simulink model "IMU_Filter_Benchmarking"  (R2026a)
settings: Solver=VariableStepAuto  StopTime=10
libraries: dspstat3 x4, simulink x3
settings Model: Creator=root  LastModifiedBy=root

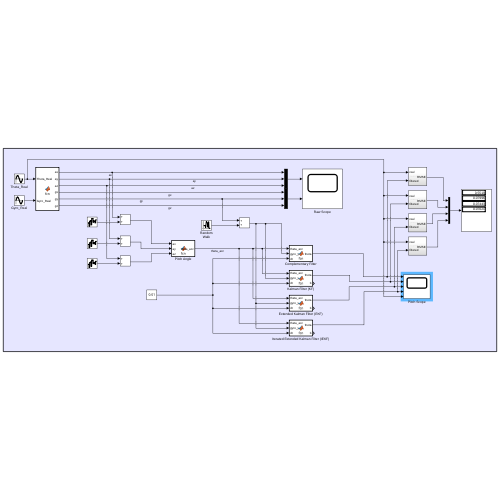
[thumbnail: Simulink's stored preview of the top-level diagram]
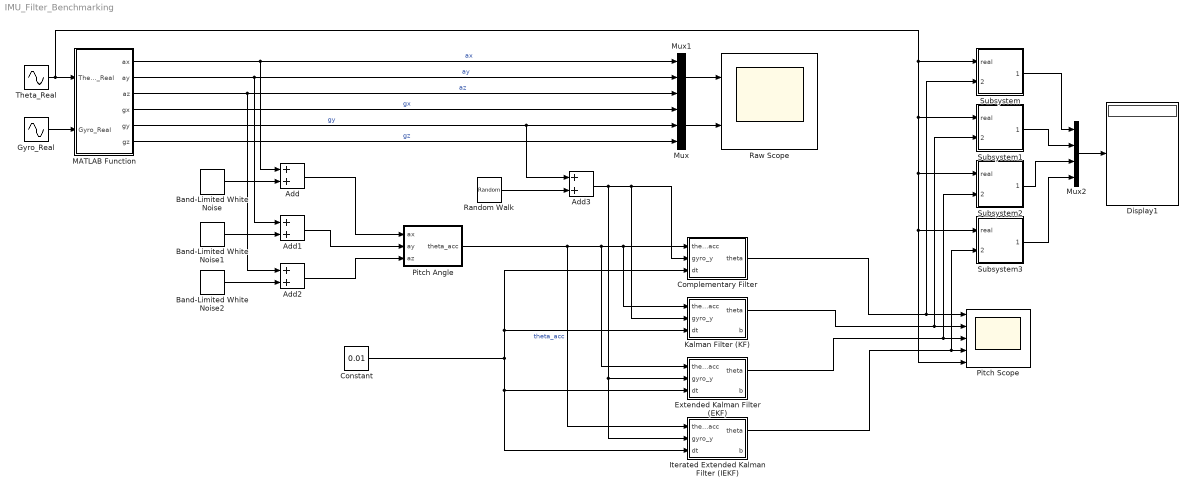
== system IMU_Filter_Benchmarking ==
  Add{,1..3} (4 alike) : Sum
  Band-Limited White Noise : simulink/Sources/Band-Limited White Noise  Cov=[0.1]  Ts=0.01  seed=[23341]
  Band-Limited White Noise1 : simulink/Sources/Band-Limited White Noise  Cov=[0.1]  Ts=0.01  seed=[24341]
  Band-Limited White Noise2 : simulink/Sources/Band-Limited White Noise  Cov=[0.1]  Ts=0.01  seed=[24741]
  Complementary Filter : MATLAB Function  TreatAsAtomicUnit=on
  Constant : Constant  Value=0.01
  Display1 : Display
  Extended Kalman Filter (EKF) : MATLAB Function  TreatAsAtomicUnit=on
  Gyro_Real : Sin  Amplitude=0.5  Phase=1.57  SampleTime=0
  Iterated Extended Kalman Filter (IEKF) : MATLAB Function  TreatAsAtomicUnit=on
  Kalman Filter (KF) : MATLAB Function  TreatAsAtomicUnit=on
  MATLAB Function : MATLAB Function  TreatAsAtomicUnit=on
  Mux : Mux  Inputs=3
  Mux1 : Mux  Inputs=3
  Mux2 : Mux
  Pitch Angle : MATLAB Function  TreatAsAtomicUnit=on
  Pitch Scope : Scope  NumInputPorts=5
      settings: ActiveDisplayYMinimum=-1.6362486288335127  ActiveDisplayYMaximum=1.8195667840554803
  Random Walk : RandomNumber  Mean=0.005  Variance=0.001  Seed=1324  SampleTime=0.01
  Raw Scope : Scope  NumInputPorts=2
      settings: ActiveDisplayYMinimum=-9.4165056943893433  ActiveDisplayYMaximum=14.411522746086121
  Subsystem : Subsystem
  Subsystem1 : Subsystem
  Subsystem2 : Subsystem
  Subsystem3 : Subsystem
  Theta_Real : Sin  Frequency=2.5  SampleTime=0
  wires:
  Iterated Extended Kalman Filter (IEKF)/1(theta) -> Subsystem3/2(filtered), Pitch Scope/4
  Extended Kalman Filter (EKF)/1(theta) -> Subsystem2/2(filtered), Pitch Scope/3
  Constant/1 -> Iterated Extended Kalman Filter (IEKF)/3(dt), Extended Kalman Filter (EKF)/3(dt), Kalman Filter (KF)/3(dt), Complementary Filter/3(dt)
  Complementary Filter/1(theta) -> Subsystem/2(filtered), Pitch Scope/1
  Mux1/1 -> Raw Scope/1
  Mux/1 -> Raw Scope/2
  MATLAB Function/1(ax) -> Mux1/1, Add/1  "ax"
  MATLAB Function/2(ay) -> Add1/1, Mux1/2  "ay"
  Pitch Angle/1(theta_acc) -> Extended Kalman Filter (EKF)/1(theta_acc), Kalman Filter (KF)/1(theta_acc), Complementary Filter/1(theta_acc), Iterated Extended Kalman Filter (IEKF)/1(theta_acc)  "theta_acc"
  Band-Limited White Noise1/1 -> Add1/2
  Band-Limited White Noise2/1 -> Add2/2
  Add3/1 -> Iterated Extended Kalman Filter (IEKF)/2(gyro_y), Extended Kalman Filter (EKF)/2(gyro_y), Kalman Filter (KF)/2(gyro_y), Complementary Filter/2(gyro_y)
  Add1/1 -> Pitch Angle/2(ay)
  Random Walk/1 -> Add3/2
  MATLAB Function/3(az) -> Add2/1, Mux1/3  "az"
  MATLAB Function/4(gx) -> Mux/1  "gx"
  MATLAB Function/6(gz) -> Mux/3  "gz"
  Kalman Filter (KF)/1(theta) -> Subsystem1/2(filtered), Pitch Scope/2
  Add/1 -> Pitch Angle/1(ax)
  MATLAB Function/5(gy) -> Add3/1, Mux/2  "gy"
  Band-Limited White Noise/1 -> Add/2
  Add2/1 -> Pitch Angle/3(az)
  Gyro_Real/1 -> MATLAB Function/2(Gyro_Real)
  Theta_Real/1 -> Subsystem/1(real), Subsystem1/1(real), Subsystem2/1(real), Subsystem3/1(real), Pitch Scope/5, MATLAB Function/1(Theta_Real)
  Subsystem/1(RMSE) -> Mux2/1
  Mux2/1 -> Display1/1
  Subsystem1/1(RMSE) -> Mux2/2
  Subsystem3/1(RMSE) -> Mux2/4
  Subsystem2/1(RMSE) -> Mux2/3

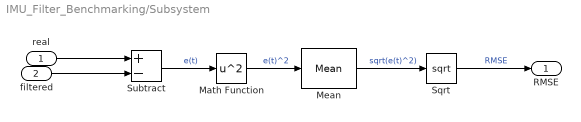
== system IMU_Filter_Benchmarking/Subsystem ==
  real : Inport
  filtered : Inport  Port=2
  Math Function : Math  Operator=square
  Mean : dspstat3/Mean  run=off  InputProcessing=Columns as channels (frame based)  reset_popup=None  directionMode=Each column  dimension=1  roiEnable=off  roiType=Rectangles  roiPortion=Entire ROI  roiOutput=Individual statistics for each ROI  roiFlag=off  roundingMode=Floor  overflowMode=off  outputDataTypeStr=Inherit: Same as accumulator  outputMin=[]  outputMax=[]  outputLastDataTypeStr=Inherit: Same as accumulator
  Sqrt : Sqrt
  Subtract : Sum  Inputs=+-
  RMSE : Outport
  wires:
  Math Function/1 -> Mean/1  "e(t)^2"
  Sqrt/1 -> RMSE/1  "RMSE"
  Mean/1 -> Sqrt/1  "sqrt(e(t)^2)"
  Subtract/1 -> Math Function/1  "e(t)"
  filtered/1 -> Subtract/2
  real/1 -> Subtract/1

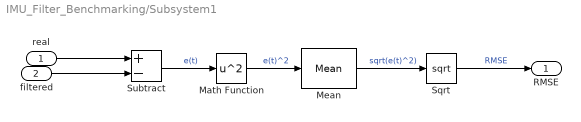
== system IMU_Filter_Benchmarking/Subsystem1 ==
  real : Inport
  filtered : Inport  Port=2
  Math Function : Math  Operator=square
  Mean : dspstat3/Mean  run=off  InputProcessing=Columns as channels (frame based)  reset_popup=None  directionMode=Each column  dimension=1  roiEnable=off  roiType=Rectangles  roiPortion=Entire ROI  roiOutput=Individual statistics for each ROI  roiFlag=off  roundingMode=Floor  overflowMode=off  outputDataTypeStr=Inherit: Same as accumulator  outputMin=[]  outputMax=[]  outputLastDataTypeStr=Inherit: Same as accumulator
  Sqrt : Sqrt
  Subtract : Sum  Inputs=+-
  RMSE : Outport
  wires:
  real/1 -> Subtract/1
  filtered/1 -> Subtract/2
  Subtract/1 -> Math Function/1  "e(t)"
  Mean/1 -> Sqrt/1  "sqrt(e(t)^2)"
  Sqrt/1 -> RMSE/1  "RMSE"
  Math Function/1 -> Mean/1  "e(t)^2"

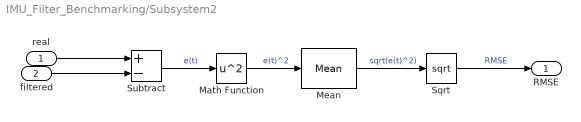
== system IMU_Filter_Benchmarking/Subsystem2 ==
  real : Inport
  filtered : Inport  Port=2
  Math Function : Math  Operator=square
  Mean : dspstat3/Mean  run=off  InputProcessing=Columns as channels (frame based)  reset_popup=None  directionMode=Each column  dimension=1  roiEnable=off  roiType=Rectangles  roiPortion=Entire ROI  roiOutput=Individual statistics for each ROI  roiFlag=off  roundingMode=Floor  overflowMode=off  outputDataTypeStr=Inherit: Same as accumulator  outputMin=[]  outputMax=[]  outputLastDataTypeStr=Inherit: Same as accumulator
  Sqrt : Sqrt
  Subtract : Sum  Inputs=+-
  RMSE : Outport
  wires:
  Math Function/1 -> Mean/1  "e(t)^2"
  Sqrt/1 -> RMSE/1  "RMSE"
  Mean/1 -> Sqrt/1  "sqrt(e(t)^2)"
  Subtract/1 -> Math Function/1  "e(t)"
  filtered/1 -> Subtract/2
  real/1 -> Subtract/1

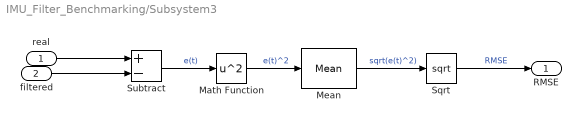
== system IMU_Filter_Benchmarking/Subsystem3 ==
  real : Inport
  filtered : Inport  Port=2
  Math Function : Math  Operator=square
  Mean : dspstat3/Mean  run=off  InputProcessing=Columns as channels (frame based)  reset_popup=None  directionMode=Each column  dimension=1  roiEnable=off  roiType=Rectangles  roiPortion=Entire ROI  roiOutput=Individual statistics for each ROI  roiFlag=off  roundingMode=Floor  overflowMode=off  outputDataTypeStr=Inherit: Same as accumulator  outputMin=[]  outputMax=[]  outputLastDataTypeStr=Inherit: Same as accumulator
  Sqrt : Sqrt
  Subtract : Sum  Inputs=+-
  RMSE : Outport
  wires:
  real/1 -> Subtract/1
  filtered/1 -> Subtract/2
  Subtract/1 -> Math Function/1  "e(t)"
  Mean/1 -> Sqrt/1  "sqrt(e(t)^2)"
  Sqrt/1 -> RMSE/1  "RMSE"
  Math Function/1 -> Mean/1  "e(t)^2"

== matlab function IMU_Filter_Benchmarking/Complementary Filter ==
  data: theta_acc input; theta output; gyro_y input; dt input
function theta = fcn(theta_acc, gyro_y, dt)
    theta_acc = double(theta_acc);
    gyro_y    = double(gyro_y);
    dt        = double(dt);

    % Set up the previous theta value
    persistent theta_prev
    if isempty(theta_prev)
        theta_prev = 0;
    end
    
    % Complementary filter w/ high-pass gyro + low-pass accelerometer
    alpha = 0.98;
    theta = alpha * (theta_prev + gyro_y * dt) + (1 - alpha) * theta_acc;
    theta_prev = theta;
end

== matlab function IMU_Filter_Benchmarking/Pitch Angle ==
  data: ax input; theta_acc output; ay input; az input
function theta_acc = fcn(ax, ay, az)
    % Calculate pitch angle in radians from static acceleration
    theta_acc = atan2(ax, sqrt(ay^2 + az^2));
end

== matlab function IMU_Filter_Benchmarking/Kalman Filter (KF) ==
  data: theta_acc input; theta output; gyro_y input; dt input; b output
function [theta, b] = fcn(theta_acc, gyro_y, dt)
    theta_acc = double(theta_acc);
    gyro_y    = double(gyro_y);
    dt        = double(dt);

    persistent x P
    if isempty(x)
        x = [0; 0];
        P = eye(2);
    end

    % --- EMPIRICAL COVARIANCE MATRICES ---
    R = 0.00000382;
    Q = [4.0e-10 , 0 ;
         0       , 1.0e-6];
    % ------------------------------------

    A = [1, -dt; 0, 1];
    B = [dt; 0];
    C = [1, 0];
    
    % Predict
    x_pred = A * x + B * gyro_y;
    P_pred = A * P * A' + Q;
    
    % Update
    K = (P_pred * C') / (C * P_pred * C' + R);
    x = x_pred + K * (theta_acc - C * x_pred);
    P = (eye(2) - K * C) * P_pred;
    
    % Clamp the angle back to [-pi, pi] interval after the state update
    x(1) = atan2(sin(x(1)), cos(x(1)));

    theta = x(1);
    b     = x(2);
end

== matlab function IMU_Filter_Benchmarking/Iterated Extended Kalman Filter (IEKF) ==
  data: theta_acc input; theta output; gyro_y input; dt input; b output
function [theta, b] = fcn(theta_acc, gyro_y, dt)
    theta_acc = double(theta_acc);
    gyro_y    = double(gyro_y);
    dt        = double(dt);

    persistent x P
    if isempty(x)
        x = [0; 0];
        P = eye(2);
    end

    % --- EMPIRICAL COVARIANCE MATRICES ---
    R = 0.00000382;
    Q = [4.0e-10 , 0 ;
         0       , 1.0e-6];
    % ------------------------------------

    A = [1, -dt; 0, 1];
    B = [dt; 0];
    
    % Predict
    x_pred = A * x + B * gyro_y;
    P_pred = A * P * A' + Q;
    
    % Iterated Update Loop
    eta = x_pred;
    num_iters = 4;
    for i = 1:num_iters
        H = [cos(eta(1)), 0];
        h_eta = sin(eta(1));
        
        K = (P_pred * H') / (H * P_pred * H' + R);
        eta = x_pred + K * (sin(theta_acc) - h_eta - H * (x_pred - eta));
    end
    
    x = eta;
    P = (eye(2) - K * H) * P_pred;
    
    % Clamp the angle back to [-pi, pi] interval after the state update
    x(1) = atan2(sin(x(1)), cos(x(1)));

    theta = x(1);
    b     = x(2);
end

== matlab function IMU_Filter_Benchmarking/Extended Kalman Filter (EKF) ==
  data: theta_acc input; theta output; gyro_y input; dt input; b output
function [theta, b] = fcn(theta_acc, gyro_y, dt)
    theta_acc = double(theta_acc);
    gyro_y    = double(gyro_y);
    dt        = double(dt);

    persistent x P
    if isempty(x)
        x = [0; 0];
        P = eye(2);
    end

    % --- EMPIRICAL COVARIANCE MATRICES ---
    R = 0.00000382;
    Q = [4.0e-10 , 0 ;
         0       , 1.0e-6];
    % ------------------------------------

    A = [1, -dt; 0, 1];
    B = [dt; 0];
    
    % Predict
    x_pred = A * x + B * gyro_y;
    P_pred = A * P * A' + Q;
    
    % Non-linear Update (Single Pass)
    H = [cos(x_pred(1)), 0];
    y_tilde = sin(theta_acc) - sin(x_pred(1));
    
    K = (P_pred * H') / (H * P_pred * H' + R);
    x = x_pred + K * y_tilde;
    P = (eye(2) - K * H) * P_pred;
    
    % Clamp the angle back to [-pi, pi] interval after the state update
    x(1) = atan2(sin(x(1)), cos(x(1)));

    theta = x(1);
    b     = x(2);
end

== matlab function IMU_Filter_Benchmarking/MATLAB Function ==
  data: ax output; ay output; az output; Theta_Real input; Gyro_Real input; gx output; gy output; gz output
function [ax, ay, az, gx, gy, gz]= fcn(Theta_Real, Gyro_Real)
    g = 9.81; % m/s2
    ax = g * sin(Theta_Real);
    ay = 0;
    az = -g * cos(Theta_Real);
    gx = 0;
    gy = Gyro_Real;
    gz = 0;
end
